simulink model "Pollution_Sensor_Simulation"  (R2025a)
settings: Solver=VariableStepAuto  StartTime=0.0  StopTime=10  RelTol=1e-3
libraries: simulink x3
settings Model: Creator=Rama  LastModifiedBy=Rama

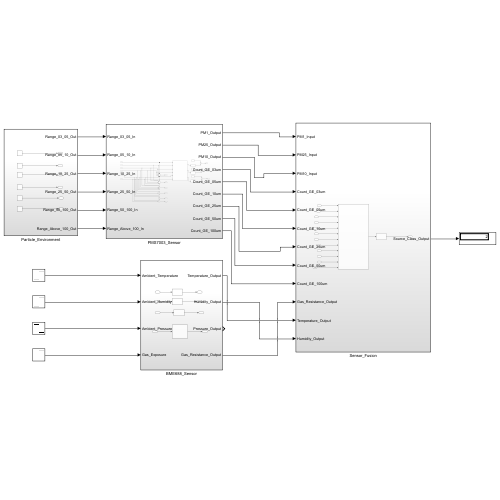
[thumbnail: Simulink's stored preview of the top-level diagram]
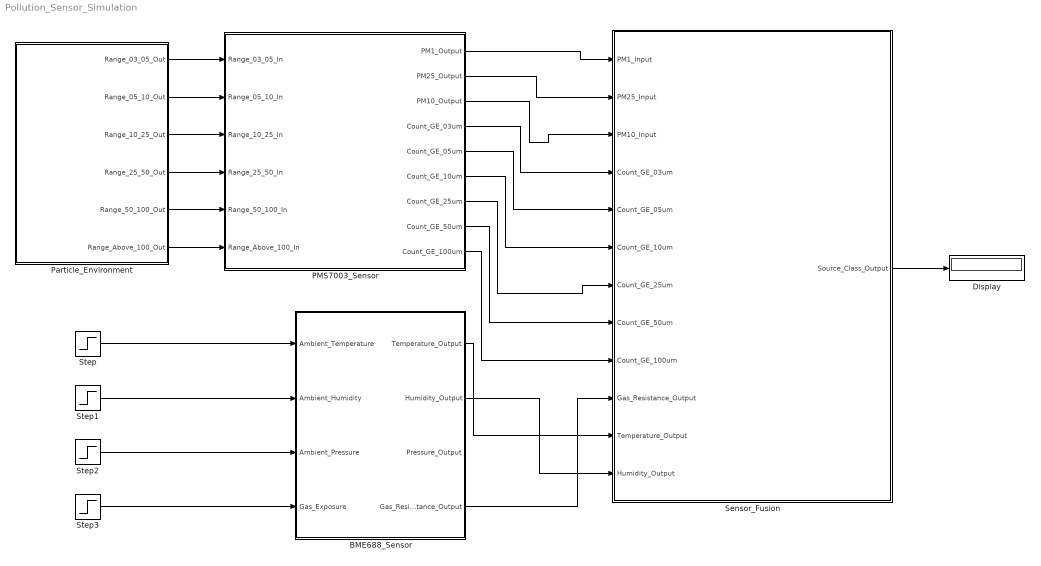
== system Pollution_Sensor_Simulation ==
  BME688_Sensor : Subsystem
  Display : Display
  PMS7003_Sensor : Subsystem
  Particle_Environment : Subsystem
  Sensor_Fusion : Subsystem
  Step : Step  Time=10  Before=28  After=28  SampleTime=0
  Step1 : Step  Time=10  Before=55  After=55  SampleTime=0
  Step2 : Step  Time=10  Before=1013  After=1010  SampleTime=0
  Step3 : Step  Time=10  Before=0.75  After=0.75  SampleTime=0
  wires:
  Particle_Environment/1(Range_03_05_Out) -> PMS7003_Sensor/1(Range_03_05_In)
  Particle_Environment/2(Range_05_10_Out) -> PMS7003_Sensor/2(Range_05_10_In)
  Particle_Environment/3(Range_10_25_Out) -> PMS7003_Sensor/3(Range_10_25_In)
  Particle_Environment/4(Range_25_50_Out) -> PMS7003_Sensor/4(Range_25_50_In)
  Particle_Environment/5(Range_50_100_Out) -> PMS7003_Sensor/5(Range_50_100_In)
  Particle_Environment/6(Range_Above_100_Out) -> PMS7003_Sensor/6(Range_Above_100_In)
  Step/1 -> BME688_Sensor/1(Ambient_Temperature)
  Step2/1 -> BME688_Sensor/3(Ambient_Pressure)
  Step1/1 -> BME688_Sensor/2(Ambient_Humidity)
  Step3/1 -> BME688_Sensor/4(Gas_Exposure)
  PMS7003_Sensor/1(PM1_Output) -> Sensor_Fusion/1(PM1_Input)
  PMS7003_Sensor/2(PM25_Output) -> Sensor_Fusion/2(PM25_Input)
  PMS7003_Sensor/3(PM10_Output) -> Sensor_Fusion/3(PM10_Input)
  PMS7003_Sensor/4(Count_GE_03um) -> Sensor_Fusion/4(Count_GE_03um)
  PMS7003_Sensor/5(Count_GE_05um) -> Sensor_Fusion/5(Count_GE_05um)
  PMS7003_Sensor/6(Count_GE_10um) -> Sensor_Fusion/6(Count_GE_10um)
  PMS7003_Sensor/7(Count_GE_25um) -> Sensor_Fusion/7(Count_GE_25um)
  PMS7003_Sensor/8(Count_GE_50um) -> Sensor_Fusion/8(Count_GE_50um)
  PMS7003_Sensor/9(Count_GE_100um) -> Sensor_Fusion/9(Count_GE_100um)
  BME688_Sensor/1(Temperature_Output) -> Sensor_Fusion/11(Temperature_Output)
  BME688_Sensor/4(Gas_Resistance_Output) -> Sensor_Fusion/10(Gas_Resistance_Output)
  BME688_Sensor/2(Humidity_Output) -> Sensor_Fusion/12(Humidity_Output)
  Sensor_Fusion/1(Source_Class_Output) -> Display/1

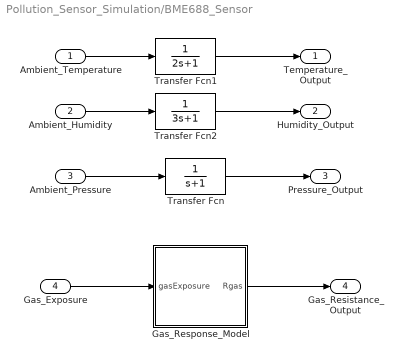
== system Pollution_Sensor_Simulation/BME688_Sensor ==
  Ambient_Temperature : Inport
  Ambient_Humidity : Inport  Port=2
  Ambient_Pressure : Inport  Port=3
  Gas_Exposure : Inport  Port=4
  Gas_Response_Model : MATLAB Function  TreatAsAtomicUnit=on
  Transfer Fcn : TransferFcn  Denominator=[1 1]
  Transfer Fcn1 : TransferFcn  Denominator=[2 1]
  Transfer Fcn2 : TransferFcn  Denominator=[3 1]
  Temperature_Output : Outport
  Humidity_Output : Outport  Port=2
  Pressure_Output : Outport  Port=3
  Gas_Resistance_Output : Outport  Port=4
  wires:
  Ambient_Pressure/1 -> Transfer Fcn/1
  Transfer Fcn/1 -> Pressure_Output/1
  Ambient_Temperature/1 -> Transfer Fcn1/1
  Transfer Fcn1/1 -> Temperature_Output/1
  Transfer Fcn2/1 -> Humidity_Output/1
  Ambient_Humidity/1 -> Transfer Fcn2/1
  Gas_Exposure/1 -> Gas_Response_Model/1(gasExposure)
  Gas_Response_Model/1(Rgas) -> Gas_Resistance_Output/1

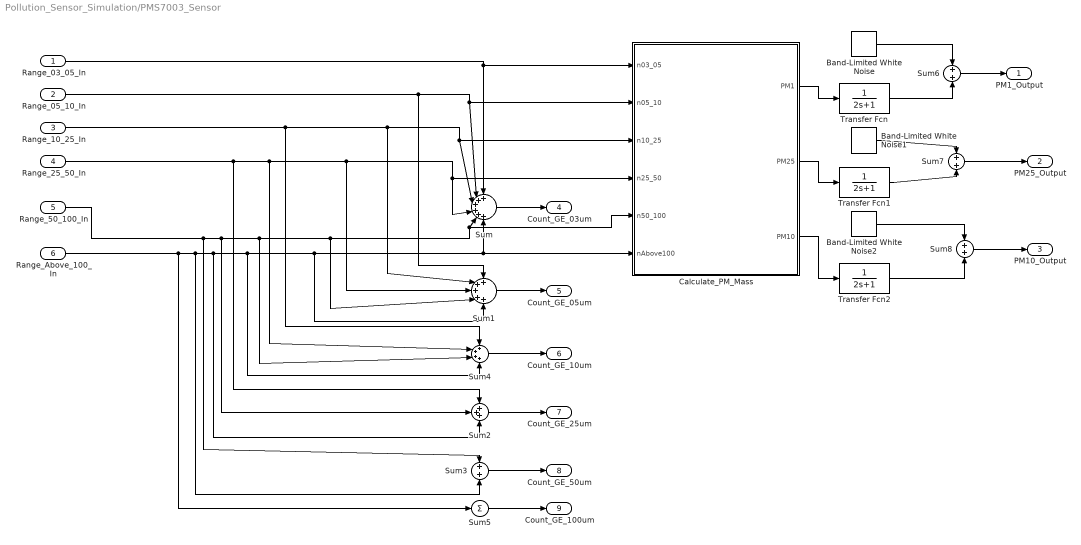
== system Pollution_Sensor_Simulation/PMS7003_Sensor ==
  Range_03_05_In : Inport
  Range_05_10_In : Inport  Port=2
  Range_10_25_In : Inport  Port=3
  Range_25_50_In : Inport  Port=4
  Range_50_100_In : Inport  Port=5
  Range_Above_100_In : Inport  Port=6
  Band-Limited White Noise : simulink/Sources/Band-Limited White Noise  Cov=[0.01]  Ts=0.1  seed=[12345]
  Band-Limited White Noise1 : simulink/Sources/Band-Limited White Noise  Cov=[0.04]  Ts=0.1  seed=[12345]
  Band-Limited White Noise2 : simulink/Sources/Band-Limited White Noise  Cov=[0.25]  Ts=0.1  seed=[12345]
  Calculate_PM_Mass : MATLAB Function  TreatAsAtomicUnit=on
  Sum : Sum  Inputs=++++++
  Sum1 : Sum  Inputs=+++++
  Sum2 : Sum  Inputs=+++
  Sum{3,6..8} (4 alike) : Sum
  Sum4 : Sum  Inputs=++++
  Sum5 : Sum  Inputs=+
  Transfer Fcn : TransferFcn  Denominator=[2 1]
  Transfer Fcn1 : TransferFcn  Denominator=[2 1]
  Transfer Fcn2 : TransferFcn  Denominator=[2 1]
  PM1_Output : Outport
  PM25_Output : Outport  Port=2
  PM10_Output : Outport  Port=3
  Count_GE_03um : Outport  Port=4
  Count_GE_05um : Outport  Port=5
  Count_GE_10um : Outport  Port=6
  Count_GE_25um : Outport  Port=7
  Count_GE_50um : Outport  Port=8
  Count_GE_100um : Outport  Port=9
  wires:
  Sum4/1 -> Count_GE_10um/1
  Sum2/1 -> Count_GE_25um/1
  Sum3/1 -> Count_GE_50um/1
  Sum5/1 -> Count_GE_100um/1
  Sum/1 -> Count_GE_03um/1
  Range_03_05_In/1 -> Calculate_PM_Mass/1(n03_05), Sum/1
  Range_05_10_In/1 -> Sum1/1, Calculate_PM_Mass/2(n05_10), Sum/2
  Range_10_25_In/1 -> Sum4/1, Sum1/2, Calculate_PM_Mass/3(n10_25), Sum/3
  Range_25_50_In/1 -> Sum4/2, Sum1/3, Calculate_PM_Mass/4(n25_50), Sum/4, Sum2/1
  Range_50_100_In/1 -> Sum4/3, Sum1/4, Calculate_PM_Mass/5(n50_100), Sum/5, Sum2/2, Sum3/1
  Range_Above_100_In/1 -> Sum5/1, Sum4/4, Sum1/5, Calculate_PM_Mass/6(nAbove100), Sum/6, Sum2/3, Sum3/2
  Sum1/1 -> Count_GE_05um/1
  Calculate_PM_Mass/1(PM1) -> Transfer Fcn/1
  Calculate_PM_Mass/2(PM25) -> Transfer Fcn1/1
  Calculate_PM_Mass/3(PM10) -> Transfer Fcn2/1
  Band-Limited White Noise/1 -> Sum6/1
  Transfer Fcn/1 -> Sum6/2
  Sum6/1 -> PM1_Output/1
  Transfer Fcn2/1 -> Sum8/2
  Sum8/1 -> PM10_Output/1
  Transfer Fcn1/1 -> Sum7/2
  Sum7/1 -> PM25_Output/1
  Band-Limited White Noise1/1 -> Sum7/1
  Band-Limited White Noise2/1 -> Sum8/1

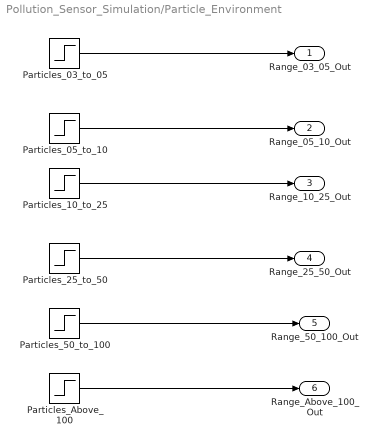
== system Pollution_Sensor_Simulation/Particle_Environment ==
  " Particles_Above_100" : Step  Time=10  Before=0.001  After=0.001  SampleTime=0
  Particles_03_to_05 : Step  Time=10  Before=150  After=150  SampleTime=0
  Particles_05_to_10 : Step  Time=10  Before=20  After=20  SampleTime=0
  Particles_10_to_25 : Step  Time=10  Before=1  SampleTime=0
  Particles_25_to_50 : Step  Time=10  Before=0.1  After=0.1  SampleTime=0
  Particles_50_to_100 : Step  Time=10  Before=0.01  After=0.01  SampleTime=0
  Range_03_05_Out : Outport
  Range_05_10_Out : Outport  Port=2
  Range_10_25_Out : Outport  Port=3
  Range_25_50_Out : Outport  Port=4
  Range_50_100_Out : Outport  Port=5
  Range_Above_100_Out : Outport  Port=6
  wires:
  Particles_03_to_05/1 -> Range_03_05_Out/1
  Particles_05_to_10/1 -> Range_05_10_Out/1
  Particles_10_to_25/1 -> Range_10_25_Out/1
  Particles_25_to_50/1 -> Range_25_50_Out/1
  Particles_50_to_100/1 -> Range_50_100_Out/1
  " Particles_Above_100"/1 -> Range_Above_100_Out/1

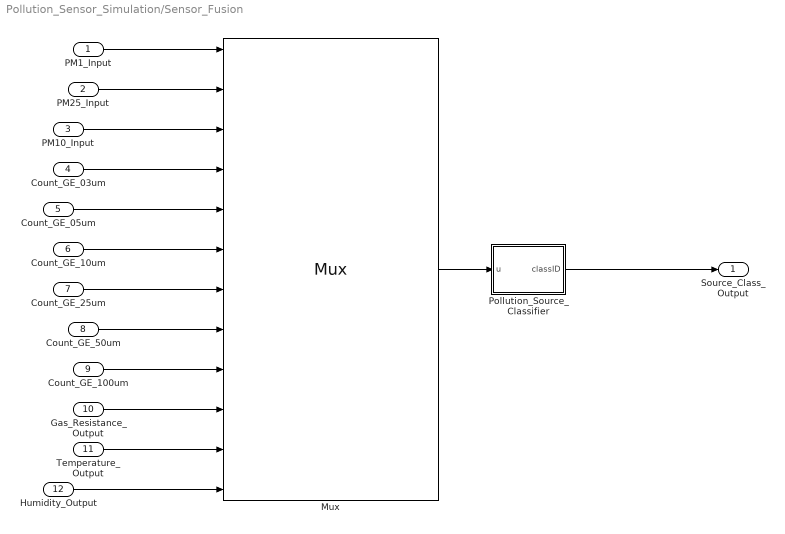
== system Pollution_Sensor_Simulation/Sensor_Fusion ==
  PM1_Input : Inport
  PM25_Input : Inport  Port=2
  PM10_Input : Inport  Port=3
  Count_GE_03um : Inport  Port=4
  Count_GE_05um : Inport  Port=5
  Count_GE_10um : Inport  Port=6
  Count_GE_25um : Inport  Port=7
  Count_GE_50um : Inport  Port=8
  Count_GE_100um : Inport  Port=9
  Gas_Resistance_Output : Inport  Port=10
  Temperature_Output : Inport  Port=11
  Humidity_Output : Inport  Port=12
  Mux : Mux  Inputs=12
  Pollution_Source_Classifier : MATLAB Function  TreatAsAtomicUnit=on
  Source_Class_Output : Outport
  wires:
  PM1_Input/1 -> Mux/1
  PM25_Input/1 -> Mux/2
  PM10_Input/1 -> Mux/3
  Count_GE_03um/1 -> Mux/4
  Count_GE_05um/1 -> Mux/5
  Count_GE_10um/1 -> Mux/6
  Count_GE_25um/1 -> Mux/7
  Count_GE_50um/1 -> Mux/8
  Count_GE_100um/1 -> Mux/9
  Gas_Resistance_Output/1 -> Mux/10
  Temperature_Output/1 -> Mux/11
  Humidity_Output/1 -> Mux/12
  Mux/1 -> Pollution_Source_Classifier/1(u)
  Pollution_Source_Classifier/1(classID) -> Source_Class_Output/1

== matlab function Pollution_Sensor_Simulation/PMS7003_Sensor/Calculate_PM_Mass ==
  data: n03_05 input; PM1 output; n05_10 input; n10_25 input; n25_50 input; n50_100 input; nAbove100 input; PM25 output; PM10 output

function [PM1, PM25, PM10] = fcn(n03_05, n05_10, n10_25, n25_50, n50_100, nAbove100)
%#codegen
% Simplified particle mass estimate.
% Inputs: number concentrations in particles/cm^3.
% Assumptions: spherical particles, density = 1000 kg/m^3.
% Illustrative model, not calibrated PMS7003 firmware.

rho = 1000; % kg/m^3

% Representative diameters for each size range, in metres.
d = [0.4, 0.75, 1.75, 3.75, 7.5, 12.0] * 1e-6;

% Particle concentrations.
n = [n03_05, n05_10, n10_25, n25_50, n50_100, nAbove100];

% Convert number concentration to particles/m^3.
N = n * 1e6;

% Estimate mass contribution from each range in micrograms/m^3.
massContribution = N .* (rho * (pi/6) .* d.^3) * 1e9;

% Cumulative PM mass estimates.
PM1  = massContribution(1) + massContribution(2);
PM25 = PM1 + massContribution(3);
PM10 = PM25 + massContribution(4) + massContribution(5);
end

== matlab function Pollution_Sensor_Simulation/BME688_Sensor/Gas_Response_Model ==
  data: gasExposure input; Rgas output

function Rgas = fcn(gasExposure)
%#codegen
% Illustrative BME688 gas-response model.
% gasExposure is a normalized test stimulus from 0 to 1.
% Output is simulated gas resistance in ohms, not calibrated data.

Rclean = 100000;  % assumed baseline resistance, ohms
Rexposed = 20000; % assumed resistance under strong exposure, ohms

u = min(max(gasExposure, 0), 1);
Rgas = Rclean - u * (Rclean - Rexposed);
end

== matlab function Pollution_Sensor_Simulation/Sensor_Fusion/Pollution_Source_Classifier ==
  data: u input; classID output

function classID = fcn(u)
%#codegen
% Decision tree trained on SYNTHETIC data.
% Input order matches the existing 12-input Mux.

x = reshape(u, 1, 12);

PM1  = x(1);
PM25 = x(2);
Rgas = x(10);
Temp = x(11);

% Reproduces the trained ClassificationTree
if PM1 < 4.51964
    classID = 1;  % Background

elseif PM1 >= 4.51964
    if Rgas < 57273.7
        if PM25 < 34.9898
            classID = 2;  % Vehicle exhaust
        elseif PM25 >= 34.9898
            if Temp < 30.6058
                classID = 5;  % Industrial emissions
            elseif Temp >= 30.6058
                classID = 3;  % Biomass burning
            else
                classID = 5;
            end
        else
            classID = 5;
        end
    elseif Rgas >= 57273.7
        classID = 4;  % Dust
    else
        classID = 4;
    end
else
    classID = 1;
end
end
